simulink model "final_project_pid"  (R2024b)
settings: Solver=ode5  StartTime=0.0  StopTime=10  FixedStep=1e-3  MaxStep=0.001  RelTol=1e-3  AbsTol=1e-5
model workspace (MATLAB code in the model file):
  | Ts=1e-3;
libraries: slpidlib x1
Description:
  | Magnetic Levitation Model
  | 
  | vrmaglev is an example showing the interaction between dynamic models in Simulink(R)
  | and virtual worlds. The Simulink model represents the HUMUSOFT(R) CE152 Magnetic Levitation
  | educational / presentation scale model. (http://www.humusoft.com/link/models)
  | 
  | The plant model is controlled by a PID controller with feed forward to cope with the nonlinearity
  | of the magnetic levitation system.
  | 
  | The position of the ball responds to the changing value of the setpoint. You can observe
  | this change not only in the Scope window, but also in a viewer window displaying
  | the virtual world. Note that the position of the ball represents the real dynamics of the system.
  | If you switch the VRML viewer to the Camera 3 viewpoint, you can observe and control the ball easier.
  | 
  | There are two possible methods of setting the ball position setpoint - using a Signal Generator
  | and visually by clicking at a desired position in the virtual reality scene.
  | 
  | In the virtual scene, a VRML sensor is defined. If you click in the space between the magnetic coil
  | and the bottom plate, VRML sensor is updated and its value is read into Simulink model using the
  | VR Source block.
settings Model: ExtModeTrigDuration=5000  ExtModeTrigLevel=0.500000  Creator=The MathWorks, Inc.  LastModifiedBy=Ali Saleh Al-Taher
settings SolverCC: AutoScaleAbsTol=off  AlgebraicLoopSolver=TrustRegion
settings DataIOCC: SaveFormat=Array  SaveOutput=off  SaveTime=off  ReturnWorkspaceOutputs=off  SignalLoggingName=logsOut
settings OptimizationCC: BlockReduction=off  BooleanDataType=off  OptimizeBlockIOStorage=off  BufferReuse=off  GlobalBufferReuse=off  ExpressionFolding=off  ExpressionDepthLimit=2147483647  LocalBlockOutputs=off  InitFltsAndDblsToZero=on  LifeSpan=inf
settings DebuggingCC: UnderspecifiedInitializationDetection=Classic  MergeDetectMultiDrivingBlocksExec=none  CheckExecutionContextPreStartOutputMsg=on  SignalResolutionControl=TryResolveAllWithWarning  MultiTaskDSMMsg=warning  MultiTaskCondExecSysMsg=none  FcnCallInpInsideContextMsg=warning  UnconnectedInputMsg=warning  UnconnectedOutputMsg=warning  UnconnectedLineMsg=warning  StateNameClashWarn=warning  SFUnexpectedBacktrackingDiag=warning  SFNoUnconditionalDefaultTransitionDiag=warning  SFExecutionAtInitializationDiag=none  ArithmeticOperatorsInVariantConditions=warning
settings HardwareCC: ProdBitPerPointer=32  ProdBitPerSizeT=32  ProdBitPerPtrDiffT=32  ProdLargestAtomicFloat=None  ProdIntDivRoundTo=Undefined  ProdEndianess=Unspecified  ProdWordSize=32  ProdHWDeviceType=32-bit Generic  TargetUnknown=on
settings ModelReferenceCC: UpdateModelReferenceTargets=IfOutOfDate  EnableRefExpFcnMdlSchedulingChecks=on  PropagateSignalLabelsOutOfModel=off
settings SFSimCC: SimUseLocalCustomCode=off  CustomCodeUndefinedFunction=UseInterfaceOnly
settings RTWCC: RetainRTWFile=on  RTWUseLocalCustomCode=off  GPUComputeCapability=3.5  DLArmComputeVersion=19.05
settings CodeAppCC: StateflowObjectComments=on
settings GRTTargetCC: TargetFcnLib=ansi_tfl_tmw.mat  TargetLangStandard=C89/C90 (ANSI)  CombineOutputUpdateFcns=off  GRTInterface=on
settings ConfigComp: CovMetricSettings=d  CovSaveCumulativeToWorkspaceVar=on  CovSaveSingleToWorkspaceVar=on  CovExternalEMLEnable=off  CovSFcnEnable=off

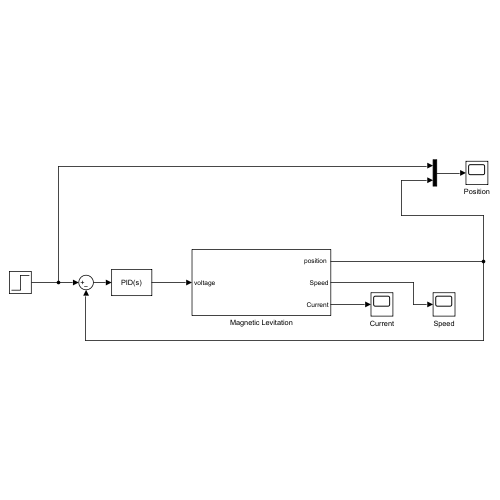
[thumbnail: Simulink's stored preview of the top-level diagram]
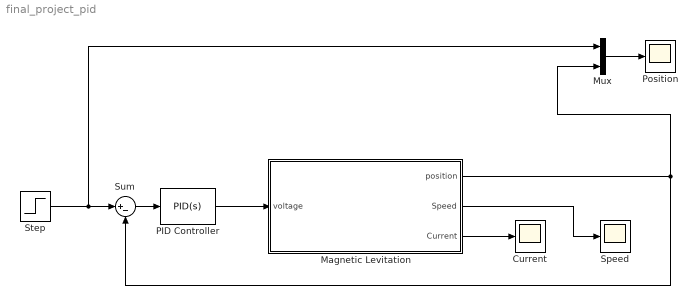
== system final_project_pid ==
  Current : Scope
  Magnetic Levitation : Subsystem
  Mux : Mux  Inputs=2
  PID Controller : slpidlib/PID Controller  Controller=PID  Form=Parallel  TimeDomain=Continuous-time  UseExternalTs=off  SampleTime=-1  IntegratorMethod=Forward Euler  FilterMethod=Forward Euler  ControllerParametersSource=internal  P=1600  I=2634  UseKiTs=off  D=244  UseExternalDerivativeSource=off  N=100  UseFilter=on  TunerSelectOption=Transfer Function Based (PID Tuner App)  InitialConditionSource=internal  InitialConditionForIntegrator=0  InitialConditionForFilter=0  DifferentiatorICPrevScaledInput=0  ExternalReset=none  TrackingMode=off  Kt=1  LimitOutput=off  SatLimitsSource=internal  UpperSaturationLimit=inf  LowerSaturationLimit=-inf  LinearizeAsGain=on  AntiWindupMode=none  Kb=1  LimitIntegrator=off  UpperIntegratorSaturationLimit=inf  LowerIntegratorSaturationLimit=-inf  POutMin=[]  POutMax=[]  IOutMin=[]  IOutMax=[]  DOutMin=[]  DOutMax=[]  NOutMin=[]  NOutMax=[]  SumOutMin=[]  SumOutMax=[]  SaturationOutMin=[]  SaturationOutMax=[]  PParamMin=[]  PParamMax=[]  IParamMin=[]  IParamMax=[]  DParamMin=[]  DParamMax=[]  NParamMin=[]  NParamMax=[]  KbParamMin=[]  KbParamMax=[]  KtParamMin=[]  KtParamMax=[]  KbOutMin=[]  KbOutMax=[]  KtOutMin=[]  KtOutMax=[]  IntegratorOutMin=[]  IntegratorOutMax=[]  FilterOutMin=[]  FilterOutMax=[]  SumI1OutMin=[]  SumI1OutMax=[]  SumI2OutMin=[]  SumI2OutMax=[]  SumI3OutMin=[]  SumI3OutMax=[]  SumI4OutMin=[]  SumI4OutMax=[]  SumDOutMin=[]  SumDOutMax=[]  DifferentiatorOutMin=[]  DifferentiatorOutMax=[]  FilterDiffOutCoefMin=[]  FilterDiffOutCoefMax=[]  ReciprocalOutMin=[]  ReciprocalOutMax=[]  SumDenOutMin=[]  SumDenOutMax=[]  SumNumOutMin=[]  SumNumOutMax=[]  DivideOutMin=[]  DivideOutMax=[]  UdiffTsProdOutMin=[]  UdiffTsProdOutMax=[]  NTsProdOutMin=[]  NTsProdOutMax=[]  UintegralTsProdOutMin=[]  UintegralTsProdOutMax=[]  UngainTsProdOutMin=[]  UngainTsProdOutMax=[]  ClampingZeroOutDataTypeStr=Inherit: Inherit via back propagation  ClampingZeroOutMin=[]  ClampingZeroOutMax=[]  FilterDenConstantOutDataTypeStr=Inherit: Inherit via back propagation  FilterDenConstantOutMin=[]  FilterDenConstantOutMax=[]  PCopyOutDataTypeStr=Inherit: Inherit via back propagation  PCopyOutMin=[]  PCopyOutMax=[]  NCopyOutDataTypeStr=Inherit: Inherit via back propagation  NCopyOutMin=[]  NCopyOutMax=[]  IntegratorContinuousStateAttributes=''  IntegratorStateMustResolveToSignalObject=off  IntegratorRTWStateStorageClass=Auto  FilterContinuousStateAttributes=''  FilterStateMustResolveToSignalObject=off  FilterRTWStateStorageClass=Auto  ParallelPVariant=InternalParameters  IdealPVariant=Disabled  IVariant=InternalParameters  DVariant=InternalParameters  IntegratorVariant=Continuous  SatVariant=Disabled  AWVariant=Passthrough  PCopyVariant=Disabled  TRVariant=Disabled  FdbkBlocksVariant=Forward  IdealPFdbkVariant=Disabled  SatFdbkVariant=Disabled  DerivativeFilterVariant=ContFilter  NVariant=InternalParameters  NCopyVariant=Disabled  FilterICVariant=InternalICsFilter  IntegratorICVariant=InternalICs  ExternalResetVariant=Disabled  TRSumVariant=Passthrough  SumFdbkVariant=Disabled  SumVariant=Sum_PID  TsampFilterVariant=InternalTs  TsampNgainVariant=Passthrough  TsampIntegralVariant=Disabled_SignalSpec  ExternalSaturationOutDataTypeStr=Inherit: Same as second input  DerivativeSourceVariant=ErrorSignal  PreIntVariant=InternalPreInt
  Position : Scope
  Speed : Scope
  Step : Step  Time=0  After=0.06  SampleTime=0
  Sum : Sum  Inputs=|+-
  wires:
  Mux/1 -> Position/1
  Magnetic Levitation/1("position ") -> Sum/2, Mux/2
  Step/1 -> Mux/1, Sum/1
  Magnetic Levitation/2(Speed) -> Speed/1
  Magnetic Levitation/3(Current) -> Current/1
  Sum/1 -> PID Controller/1
  PID Controller/1 -> Magnetic Levitation/1(voltage)

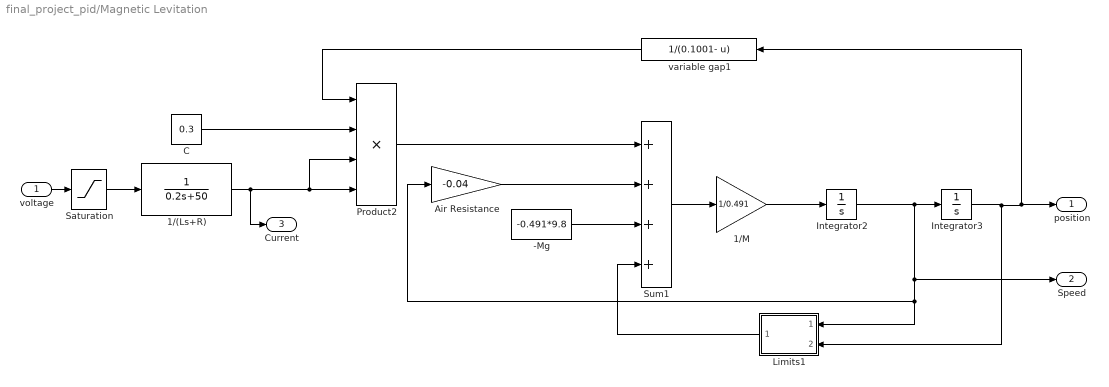
== system final_project_pid/Magnetic Levitation ==
  voltage : Inport
  -Mg : Constant  Value=-0.491*9.8
  1/(Ls+R) : TransferFcn  Denominator=[0.2 50]
  1/M : Gain  Gain=1/0.491
  Air Resistance : Gain  Gain=-0.04
  C : Constant  Value=0.3
  Integrator2 : Integrator  LowerSaturationLimit=0
  Integrator3 : Integrator  InitialCondition=0.0001  LimitOutput=on  UpperSaturationLimit=0.1  LowerSaturationLimit=0
  Limits1 : Subsystem
      mask Display: disp('LIMIT')
  Product2 : Product  Inputs=4
  Saturation : Saturate  UpperLimit=200  LowerLimit=0  ZeroCross=off
  Sum1 : Sum  Inputs=++++
  variable gap1 : Fcn  Expr=1/(0.1001- u)
  "position " : Outport  VectorParamsAs1DForOutWhenUnconnected=off
  Speed : Outport  Port=2  VectorParamsAs1DForOutWhenUnconnected=off
  Current : Outport  Port=3  VectorParamsAs1DForOutWhenUnconnected=off
  wires:
  -Mg/1 -> Sum1/3
  1/(Ls+R)/1 -> Current/1, Product2/3, Product2/4
  Sum1/1 -> 1/M/1
  Saturation/1 -> 1/(Ls+R)/1
  Integrator2/1 -> Speed/1, Limits1/1(velocity), Air Resistance/1, Integrator3/1
  Limits1/1(force) -> Sum1/4
  C/1 -> Product2/2
  Product2/1 -> Sum1/1
  1/M/1 -> Integrator2/1
  Air Resistance/1 -> Sum1/2
  variable gap1/1 -> Product2/1
  voltage/1 -> Saturation/1
  Integrator3/1 -> Limits1/2(position), "position "/1, variable gap1/1

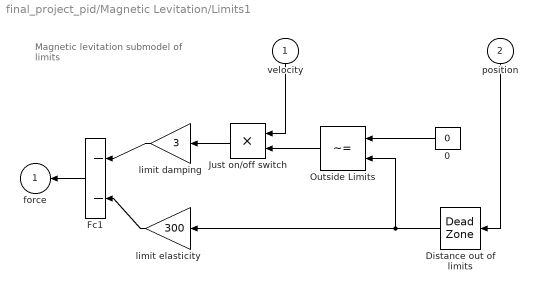
== system final_project_pid/Magnetic Levitation/Limits1 ==
  note: Magnetic levitation
      | submodel of limits
  velocity : Inport
  position : Inport  Port=2
  0 : Constant  Value=0
  Distance out of limits : DeadZone  LowerValue=0.0002  UpperValue=0.0998  ZeroCross=off
  Fc1 : Sum  Inputs=--  InputSameDT=on  SaturateOnIntegerOverflow=on  OutDataTypeStr=Inherit: Same as first input
  "Just on/off switch " : Product  InputSameDT=on  SaturateOnIntegerOverflow=on  OutDataTypeStr=Inherit: Same as first input
  Outside Limits : RelationalOperator  Operator=~=
  limit damping : Gain  Gain=3  SaturateOnIntegerOverflow=on  OutDataTypeStr=Inherit: Same as input  ParamDataTypeStr=Inherit: Same as input
  limit elasticity : Gain  Gain=300  SaturateOnIntegerOverflow=on  OutDataTypeStr=Inherit: Same as input  ParamDataTypeStr=Inherit: Same as input
  force : Outport  VectorParamsAs1DForOutWhenUnconnected=off
  wires:
  Distance out of limits/1 -> Outside Limits/2, limit elasticity/1
  limit damping/1 -> Fc1/1
  limit elasticity/1 -> Fc1/2
  Outside Limits/1 -> "Just on/off switch "/2
  0/1 -> Outside Limits/1
  "Just on/off switch "/1 -> limit damping/1
  velocity/1 -> "Just on/off switch "/1
  Fc1/1 -> force/1
  position/1 -> Distance out of limits/1
